simulink model "turbo_controller"  (R2025a)
settings: Solver=FixedStepAuto  StartTime=0.0  StopTime=inf  FixedStep=0.001  RelTol=1e-3
PostLoadFcn:
  | % 自动定位同目录CubeMX文件；不需要外部初始化脚本。
  | codertarget.data.setParameterValue('turbo_controller','STM32CubeMX.ProjectFile',fullfile(fileparts(get_param('turbo_controller','FileName')),'turbo_f407.ioc'));
InitFcn:
  | % 中文说明：按原控制器字段与类型创建三组接口总线；控制参数已内嵌。
  | tc_names=["EValve_Cycle" "EValve_Open" "Eblast_Cycle" "Eblast_Open" "Motor_Cycle" "Motor_Open" "EValve_Enable" "Eblast_Enable" "Motor_Enable" "SWO_Firework" "SWO_BleedAir" "EngineState" "Flag_ECUReset_Clear" "Flag_ECUReset_Save" "Flag_Reset_Enable" "Accelerator" "Nc_dem" "Nc"]; tc_types=["uint16" "uint16" "uint16" "uint16" "uint16" "uint16" "uint8" "uint8" "uint8" "uint8" "uint8" "uint8" "uint8" "uint8" "uint8" "single" "single" "single"];
  | for tc_k=1:numel(tc_names)
  |  tc_e(tc_k)=Simulink.BusElement; tc_e(tc_k).Name=char(tc_names(tc_k)); tc_e(tc_k).DataType=char(tc_types(tc_k));
  | end
  | EngineControl_Out=Simulink.Bus; EngineControl_Out.DataScope='Exported'; EngineControl_Out.Elements=tc_e;
  | clear tc_e tc_names tc_types tc_k
  | tc_names=["savedata1" "savedata2" "savedata3" "savedata4" "savedata5" "savedata6" "savedata7" "savedata8" "savedata9" "savedata10" "savedata11" "savedata12" "savedata13" "savedata14" "savedata15" "savedata16" "savedata17" "savedata18" "savedata19" "savedata20" "savedata21" "savedata22" "savedata23" "savedata24" "savedata25"]; tc_types=["single" "single" "single" "single" "single" "single" "single" "single" "single" "single" "single" "single" "single" "single" "single" "single" "single" "single" "single" "single" "single" "single" "single" "single" "single"];
  | for tc_k=1:numel(tc_names)
  |  tc_e(tc_k)=Simulink.BusElement; tc_e(tc_k).Name=char(tc_names(tc_k)); tc_e(tc_k).DataType=char(tc_types(tc_k));
  | end
  | SaveData_Out=Simulink.Bus; SaveData_Out.DataScope='Exported'; SaveData_Out.Elements=tc_e;
  | clear tc_e tc_names tc_types tc_k
  | tc_names=["senddata1" "senddata2" "senddata3" "senddata4" "senddata5" "senddata6" "senddata7" "senddata8" "senddata9" "senddata10" "senddata11" "senddata12" "senddata13" "senddata14" "senddata15" "senddata16" "senddata17" "senddata18" "senddata19" "senddata20" "senddata21" "senddata22" "senddata23" "senddata24" "senddata25" "senddata26" "senddata27" "senddata28" "senddata29"]; tc_types=["uint8" "uint8" "uint8" "uint8" "uint8" "uint8" "uint8" "uint8" "uint8" "uint8" "uint8" "uint8" "uint8" "uint8" "uint8" "uint8" "uint8" "uint8" "uint8" "uint8" "uint8" "uint8" "uint8" "uint8" "uint8" "uint8" "uint8" "uint8" "uint8"];
  | for tc_k=1:numel(tc_names)
  |  tc_e(tc_k)=Simulink.BusElement; tc_e(tc_k).Name=char(tc_names(tc_k)); tc_e(tc_k).DataType=char(tc_types(tc_k));
  | end
  | SendData_Out=Simulink.Bus; SendData_Out.DataScope='Exported'; SendData_Out.Elements=tc_e;
  | clear tc_e tc_names tc_types tc_k
  | 
  | % 以下为接口中文说明；只设置描述，不改变数值或数据类型。
  | EngineControl_Out.Description='执行控制输出（阀、电机、点火、状态及复位请求）';
  | tc_cn=["EValve_Cycle（主油阀周期计数（每计数2毫秒））" "EValve_Open（主油阀开通计数（每计数2毫秒））" "Eblast_Cycle（副油阀周期计数（每计数2毫秒））" "Eblast_Open（副油阀开通计数（每计数2毫秒））" "Motor_Cycle（起动电机周期计数）" "Motor_Open（起动电机开通计数）" "EValve_Enable（主油阀驱动使能）" "Eblast_Enable（副油阀驱动使能）" "Motor_Enable（起动电机使能）" "SWO_Firework（点火器使能（1开））" "SWO_BleedAir（引气阀使能（1开））" "EngineState（发动机状态）" "Flag_ECUReset_Clear（清除复位恢复状态请求）" "Flag_ECUReset_Save（保存复位恢复数据请求）" "Flag_Reset_Enable（处理器软件复位请求）" "Accelerator（油门／油泵给定控制量）" "Nc_dem（控制目标转速）" "Nc（发动机反馈转速（转每分））"];
  | tc_elements=EngineControl_Out.Elements;
  | for tc_k=1:numel(tc_cn)
  |  tc_elements(tc_k).Description=char(tc_cn(tc_k));
  | end
  | EngineControl_Out.Elements=tc_elements;
  | clear tc_cn tc_elements tc_k
  | SaveData_Out.Description='25项运行记录；字段含义按当前模型数据来源解释';
  | tc_cn=["savedata1（指令回显记录）" "savedata2（入口总温记录（℃））" "savedata3（电源电压记录）" "savedata4（排气温度记录（℃））" "savedata5（标定燃油压力记录）" "savedata6（副油阀占空比记录（％））" "savedata7（主油阀占空比记录（％））" "savedata8（温度修正转速记录）" "savedata9（开关输出及反馈位域）" "savedata10（物理转速记录）" "savedata11（油泵目标给定原始值）" "savedata12（起动电机占空比记录（％））" "savedata13（发动机状态码记录）" "savedata14（故障告警位域记录）" "savedata15（模型记录帧序号）" "savedata16（处理器温度记录（℃））" "savedata17（装订转速记录（沿用旧电源字段名））" "savedata18（导航高度记录）" "savedata19（飞行空速记录）" "savedata20（主阀旧记录位（恒零保留））" "savedata21（第21项保留记录（恒零））" "savedata22（保留记录项22）" "savedata23（保留记录项23）" "savedata24（保留记录项24）" "savedata25（保留记录项25）"];
  | tc_elements=SaveData_Out.Elements;
  | for tc_k=1:numel(tc_cn)
  |  tc_elements(tc_k).Description=char(tc_cn(tc_k));
  | end
  | SaveData_Out.Elements=tc_elements;
  | clear tc_cn tc_elements tc_k
  | SendData_Out.Description='29字段回传及外设命令接口；板端上位机帧只取第3至27字段';
  | tc_cn=["senddata1（回传发送允许标志（不直接上线路））" "senddata2（回传载荷长度25字节）" "senddata3（回传指令回显字节）" "senddata4（总温编码字节（℃＋80））" "senddata5（电源电压编码字节）" "senddata6（排温编码高字节）" "senddata7（排温编码低字节）" "senddata8（燃油压力编码高字节）" "senddata9（燃油压力编码低字节）" "senddata10（副油阀占空比字节（％））" "senddata11（主油阀占空比字节（％））" "senddata12（修正转速编码高字节）" "senddata13（修正转速编码低字节）" "senddata14（驱动及反馈状态位域）" "senddata15（物理转速编码高字节）" "senddata16（物理转速编码低字节）" "senddata17（油泵目标给定高字节（串口二使用））" "senddata18（油泵目标给定低字节（串口二使用））" "senddata19（起动电机占空比命令（串口一使用））" "senddata20（发动机状态码字节）" "senddata21（故障告警位域字节）" "senddata22（帧序号占位（板端另行填写））" "senddata23（处理器温度编码（℃＋50））" "senddata24（控制目标转速编码高字节）" "senddata25（控制目标转速编码低字节）" "senddata26（占位字节（板端改填实测泵速高字节））" "senddata27（占位字节（板端改填实测泵速低字节））" "senddata28（装订转速高字节（本板未发送））" "senddata29（装订转速低字节（本板未发送））"];
  | tc_elements=SendData_Out.Elements;
  | for tc_k=1:numel(tc_cn)
  |  tc_elements(tc_k).Description=char(tc_cn(tc_k));
  | end
  | SendData_Out.Elements=tc_elements;
  | clear tc_cn tc_elements tc_k
  | 
  | 
  | % FRAM模块化事务：接口类型和上电初始状态，随模型保存，无外部初始化文件。
  | clear FM_elements
  | FM_elements(1)=Simulink.BusElement;FM_elements(1).Name='phase';FM_elements(1).DataType='uint8';FM_elements(1).Dimensions=[1 1];FM_elements(1).Description='phase（当前事务阶段）';
  | FM_elements(2)=Simulink.BusElement;FM_elements(2).Name='a';FM_elements(2).DataType='uint8';FM_elements(2).Dimensions=[64 1];FM_elements(2).Description='a（启动时缓存的首区64字节）';
  | FM_elements(3)=Simulink.BusElement;FM_elements(3).Name='active';FM_elements(3).DataType='uint16';FM_elements(3).Dimensions=[1 1];FM_elements(3).Description='active（当前有效记录区地址）';
  | FM_elements(4)=Simulink.BusElement;FM_elements(4).Name='generation';FM_elements(4).DataType='uint32';FM_elements(4).Dimensions=[1 1];FM_elements(4).Description='generation（当前有效记录代号）';
  | FM_elements(5)=Simulink.BusElement;FM_elements(5).Name='record';FM_elements(5).DataType='uint8';FM_elements(5).Dimensions=[64 1];FM_elements(5).Description='record（本次冻结的待写记录）';
  | FM_elements(6)=Simulink.BusElement;FM_elements(6).Name='addr';FM_elements(6).DataType='uint16';FM_elements(6).Dimensions=[1 1];FM_elements(6).Description='addr（本次备用写入地址）';
  | FM_elements(7)=Simulink.BusElement;FM_elements(7).Name='lastSave';FM_elements(7).DataType='single';FM_elements(7).Dimensions=[1 1];FM_elements(7).Description='lastSave（上次开始保存的秒数）';
  | FM_elements(8)=Simulink.BusElement;FM_elements(8).Name='lastState';FM_elements(8).DataType='uint8';FM_elements(8).Dimensions=[1 1];FM_elements(8).Description='lastState（上次保存时的发动机状态）';
  | FM_elements(9)=Simulink.BusElement;FM_elements(9).Name='boot';FM_elements(9).DataType='boolean';FM_elements(9).Dimensions=[1 1];FM_elements(9).Description='boot（启动记录是否允许恢复）';
  | FM_elements(10)=Simulink.BusElement;FM_elements(10).Name='consumed';FM_elements(10).DataType='boolean';FM_elements(10).Dimensions=[1 1];FM_elements(10).Description='consumed（本次启动恢复通知是否已发送）';
  | FM_elements(11)=Simulink.BusElement;FM_elements(11).Name='payload';FM_elements(11).DataType='uint8';FM_elements(11).Dimensions=[20 1];FM_elements(11).Description='payload（当前20字节恢复内容）';
  | ... (+35 lines)
model workspace (MAT data in the model file):
  CRC16_Table_Reference = [0 4129 8258 12387 16516 20645 24774 28903 33032 37161 41290 45419 ... (256 elements, 256x1)]
  PE_Kaer = [0.15402 0.15402 0.12264 0.10076 0.09481 0.07601 0.07111 0.0569 0.05198 0.04926 0.05308 0.04325 ... (13 elements, 1x13)]
  PE_Nr = [21.2982 61.4260372 67.7475458 72.7394382 76.845934 80.6988798 83.8449282 86.6491912 88.9382406 89.178606 91.1938214 93.4068058 ... (13 elements, 1x13)]
  PE_Pump_Translate = 33.5999984741
  PE_RotaSpeed_Translate = 860
  PE_Taer = [0.4939154 0.4939154 0.40780982 0.34066978 0.31622756 0.30405716 0.34300244 0.26785022 0.37393554 0.23914836 0.44563948 0.31044662 ... (13 elements, 1x13)]
  PF_ACCFULLRANGE = 3360
  PF_Flag_ECUReset = 0
  PF_Flag_rx_suc = 1
  PF_Gear_Info = [40000; 45000; 50000; 55000; 57000; 59000; 60000; 61000; 61000; 61000; 61000; 61000]
  PF_K_TiaoJie = 1
  PF_Kpu = 10
  PF_MySet_Rxdata = [0 0 0 0 0 0 0 0 0 0 0 0 ... (50 elements, 50x1)]
  PF_MyUsart1_Rxdata = [0 0 0 0 0 0 0 0 0 0 0 0 ... (50 elements, 50x1)]
  PF_MyUsart2_Rxdata = [0 0 0 0 0 0 0 0 0 0 0 0 ... (50 elements, 50x1)]
  PF_Reset_Information = [0 0 0 0 0 0 0 0 0 0 0 0 ... (20 elements, 20x1)]
  PF_Sensor_X1_T4 = [0 4095]
  PF_Sensor_X2_T4 = [0 1.66666698456]
  PF_Sensor_X3_T4 = [0 504 999 1497 2010 2529 3051 3568 4076 4571 4959]
  PF_Sensor_X_P2 = [0.5 3]
  PF_Sensor_X_Poil = [0.5 3]
  PF_Sensor_X_T1t = [-50 300]
  PF_Sensor_X_Vpower = [0 3]
  PF_Sensor_X_Vpump = [0 3]
  PF_Sensor_Y1_T4 = [0 3]
  PF_Sensor_Y2_T4 = [0 5000]
  PF_Sensor_Y3_T4 = [0 100 200 300 400 500 600 700 800 900 980]
  PF_Sensor_Y_P2 = [0 1000]
  PF_Sensor_Y_Poil = [0 1000]
  PF_Sensor_Y_T1t = [-50 300]
  PF_Sensor_Y_Vpower = [0 33]
  PF_Sensor_Y_Vpump = [0 33]
  PG_CtrlMode_CloseLoop : mpt.Parameter (value not decoded)
  PG_CtrlMode_ManualAcc : mpt.Parameter (value not decoded)
  PG_CtrlMode_Origin : mpt.Parameter (value not decoded)
  PG_CtrlMode_Start : mpt.Parameter (value not decoded)
  PG_CtrlMode_Stop : mpt.Parameter (value not decoded)
  PG_ES_Clp : mpt.Parameter (value not decoded)
  PG_ES_EngStart : mpt.Parameter (value not decoded)
  PG_ES_Manual : mpt.Parameter (value not decoded)
  PG_ES_Origin : mpt.Parameter (value not decoded)
  PG_ES_Stop : mpt.Parameter (value not decoded)
  PG_Instr_BleedAirSet : mpt.Parameter (value not decoded)
  PG_Instr_CloseLoop : mpt.Parameter (value not decoded)
  PG_Instr_ECUReSet : mpt.Parameter (value not decoded)
  PG_Instr_EValveSet : mpt.Parameter (value not decoded)
  PG_Instr_EblastSet : mpt.Parameter (value not decoded)
  PG_Instr_Erase : mpt.Parameter (value not decoded)
  PG_Instr_FireWorkSet : mpt.Parameter (value not decoded)
  PG_Instr_ManualPlus : mpt.Parameter (value not decoded)
  PG_Instr_ManualrReduce : mpt.Parameter (value not decoded)
  PG_Instr_MotorSet : mpt.Parameter (value not decoded)
  PG_Instr_OilSet : mpt.Parameter (value not decoded)
  PG_Instr_SelfCheck : mpt.Parameter (value not decoded)
  PG_Instr_Start : mpt.Parameter (value not decoded)
  PG_Instr_Stop : mpt.Parameter (value not decoded)
  PG_Instr_StopZero : Simulink.Parameter (value not decoded)
  PG_Location_Air : Simulink.Parameter (value not decoded)
  PG_Location_Gnd : Simulink.Parameter (value not decoded)
  PG_ServoCtrlMode_CloseLoop : Simulink.Parameter (value not decoded)
  PG_ServoCtrlMode_CloseLoopMax : Simulink.Parameter (value not decoded)
  PG_ServoCtrlMode_CloseLoopMin : Simulink.Parameter (value not decoded)
  PG_ServoCtrlMode_ManualAcc : Simulink.Parameter (value not decoded)
  PG_ServoCtrlMode_ManualAccMax : Simulink.Parameter (value not decoded)
  PG_ServoCtrlMode_ManualAccMin : Simulink.Parameter (value not decoded)
  PG_SpeedDot_Permit : Simulink.Parameter (value not decoded)
  PL_EngineModel_Actuator = [0 10 100]
  PL_EngineModel_EngineStar_Press_P2 = [1013 1098.4 1099.144828 1099.931034 1103.613793 1162.662069 1143.793103 1131.006897 1123.186207 1117.6 1114 1111.806897 ... (127 elements, 1x127)]
  PL_EngineModel_EngineStar_RotaSpeed = [200 2000 9584 9660 10220 10240 10260 10288 10308 10368 10380 10408 ... (127 elements, 1x127)]
  PL_EngineModel_EngineStar_Temp_Exhaust = [128 129 129.1 130 131 131.1 132 133 134 134.1 135 135.1 ... (127 elements, 1x127)]
  PL_EngineModel_EngineStar_Time = [0.05 0.1 0.15 0.2 0.25 0.3 0.35 0.4 0.45 0.5 0.55 0.6 ... (127 elements, 1x127)]
  PL_EngineModel_IdleAbove_Nr = [0 21.2982 61.4260372 67.7475458 72.7394382 76.845934 80.6988798 83.8449282 86.6491912 88.9382406 89.178606 91.1938214 ... (14 elements, 1x14)]
  PL_EngineModel_IdleAbove_P2r = [0.986923266716 1.57907722675 1.81593881076 1.99358499877 2.23044658278 2.43770046879 2.65482358747 2.84233900814 3.03972366149 3.18776215149 3.25684678016 3.3950160375 ... (14 elements, 1x14)]
  PL_EngineModel_IdleAbove_Tempr = [0.0536001429337 1.07200285867 1.63301768805 1.63659103091 1.66875111667 1.72592460247 1.77595140254 1.86171163123 1.95461854565 2.03323208862 2.03323208862 2.13685903162 ... (14 elements, 1x14)]
  PL_EngineModel_IdleAbove_Ter = [0.42434128 0.42434128 0.42434128 0.30669408 0.23570008 0.22150128 0.1997974 0.23803274 0.16115638 0.24279948 0.13600422 0.31308354 ... (14 elements, 1x14)]
  PL_EngineModel_IdleAbove_Wfr = [0 10.142 23.8337 27.8905 31.9473 36.0041 40.0609 44.1177 48.1745 52.2313 52.7384 56.7952 ... (14 elements, 1x14)]
  PL_EngineModel_Press_P2 = [400 400 400 400 400 400 400 400 400 400]
  PL_EngineModel_Rotaspeed = [0 20000 96400]
  PL_EngineModel_Temp_Exhaust = [500 500 500 500 500 500 500 500 500 500]
  PL_Kaer = [0.1 0.1 0.1 0.1 0.1 0.1]
  PL_Nr = [50 60 70 80 90 100]
  PL_Taer = [0.1 0.1 0.1 0.1 0.1 0.1]
  Sig : Simulink.Signal (value not decoded)
  Ts_ms : Simulink.Parameter (value not decoded)
  false : Simulink.Parameter (value not decoded)
  true : Simulink.Parameter (value not decoded)
symbols that are objects in the model workspace (value not decoded): PG_CtrlMode_CloseLoop, PG_CtrlMode_ManualAcc, PG_CtrlMode_Origin, PG_CtrlMode_Start, PG_CtrlMode_Stop, PG_ES_Clp, PG_ES_EngStart, PG_ES_Manual, PG_ES_Origin, PG_ES_Stop, PG_Instr_BleedAirSet, PG_Instr_CloseLoop, PG_Instr_EblastSet, PG_Instr_ECUReSet, PG_Instr_Erase, PG_Instr_EValveSet, PG_Instr_FireWorkSet, PG_Instr_ManualPlus, PG_Instr_ManualrReduce, PG_Instr_MotorSet, PG_Instr_OilSet, PG_Instr_SelfCheck, PG_Instr_Start, PG_Instr_Stop, PG_Instr_StopZero, PG_ServoCtrlMode_CloseLoop, PG_ServoCtrlMode_CloseLoopMax, PG_ServoCtrlMode_CloseLoopMin, PG_ServoCtrlMode_ManualAcc, PG_ServoCtrlMode_ManualAccMax, PG_ServoCtrlMode_ManualAccMin, Ts_ms
libraries: simulink x97, stm32blockslib x10, stm32f4xxblockslib x8
(part 26 of 26)

== stateflow chart turbo_controller/CLM/ClpControl/Aim__Parameter_Calculate/Aim_AccMaxMin_Cal1/HoldFirst/M_Rate_Limiter ==
  note: 目标转速怎样逐次接近装订值
      |
      | 输入Nc_Initial是进入时锁存的反馈转速，S_Dem_SpeedLoad是上位机要求。第一次先令受限目标等于
      | 初值，再根据目标在初值上方还是下方，记住上升或下降阶段。
      |
      | 上升时每次图表调用加140；下降时每次减100。若本次跨过装订目标，就直接取装订目标并进入跟随阶
      | 段。后续需求再次改变，仍按同样上升/下降步长逼近。
      | 可写成上升：新目标=min(旧目标+140,需求)；下降：新目标=max(旧目标-100,需求)。
      |
      | 例如40000升到40500，输出约40140、40280、40420、40500，最后一步不是40560。每次调用的140/100
      | 是转速增量，不是每秒的变化率；按20 ms有效调用折算才有每秒意义。
      |
      | 结果送父级形成Nc_dem，不直接改变实际转速，也不直接生成油泵给定。
  (default) -> (junction 26)
    settings: description=无附加条件的迁移路径，执行次序1；沿本图当前连接推进。
  (junction 26) -> (junction 3) [order 1] : [Start_A/*起动阶段或中间量编号*/== true/*真值*/]
    settings: description=本路径的判据/动作：[Start_A== true]。执行次序1；条件成立才执行本箭头动作。
  (junction 3) -> (junction 86) [order 1] : [S_Dem_SpeedLoad/*目标需求速度或转速负载或装订值*/>=Nc_Initial/*控制器转速变量初始*/]
    settings: description=本路径的判据/动作：[S_Dem_SpeedLoad>=Nc_Initial]。执行次序1；条件成立才执行本箭头动作。
  (junction 26) -> (junction 43) [order 2]
    settings: description=无附加条件的迁移路径，执行次序2；沿本图当前连接推进。
  (junction 3) -> (junction 55) [order 2] : {Start_A/*起动阶段或中间量编号*/ = false/*假值*/;
      | S_Dem_SpeedLoad_Limiter/*目标需求速度或转速负载或装订值限制器*/=Nc_Initial/*控制器转速变量初始*/;
      | Start_C/*起动条件输入或阶段编号*/= true/*真值*/;}
    settings: description=本路径的判据/动作：{Start_A = false; S_Dem_SpeedLoad_Limiter=Nc_Initial; Start_C= true;}。执行次序2；条件成立才执行本箭头动作。
  (junction 86) -> (junction 88) : {Start_A/*起动阶段或中间量编号*/ = false/*假值*/;
      | S_Dem_SpeedLoad_Limiter/*目标需求速度或转速负载或装订值限制器*/=Nc_Initial/*控制器转速变量初始*/;
      | Start_B/*起动阶段或中间量编号*/= true/*真值*/;}
    settings: description=本路径的判据/动作：{Start_A = false; S_Dem_SpeedLoad_Limiter=Nc_Initial; Start_B= true;}。执行次序1；条件成立才执行本箭头动作。
  (junction 55) -> (junction 43)
    settings: description=无附加条件的迁移路径，执行次序1；沿本图当前连接推进。
  (junction 88) -> (junction 55)
    settings: description=无附加条件的迁移路径，执行次序1；沿本图当前连接推进。
  (junction 43) -> (junction 71)
    settings: description=无附加条件的迁移路径，执行次序1；沿本图当前连接推进。
  (junction 71) -> (junction 94) [order 1] : [Start_B/*起动阶段或中间量编号*/== true/*真值*/]
    settings: description=本路径的判据/动作：[Start_B== true]。执行次序1；条件成立才执行本箭头动作。
  (junction 71) -> (junction 106) [order 2]
    settings: description=无附加条件的迁移路径，执行次序2；沿本图当前连接推进。
  (junction 94) -> (junction 95) : {S_Dem_SpeedLoad_Limiter/*目标需求速度或转速负载或装订值限制器*/=S_Dem_SpeedLoad_Limiter/*目标需求速度或转速负载或装订值限制器*/+140.0;}
    settings: description=本路径的判据/动作：{S_Dem_SpeedLoad_Limiter=S_Dem_SpeedLoad_Limiter+140.0;}。执行次序1；条件成立才执行本箭头动作。
  (junction 95) -> (junction 99) [order 1] : [S_Dem_SpeedLoad_Limiter/*目标需求速度或转速负载或装订值限制器*/>=S_Dem_SpeedLoad/*目标需求速度或转速负载或装订值*/]
    settings: description=本路径的判据/动作：[S_Dem_SpeedLoad_Limiter>=S_Dem_SpeedLoad]。执行次序1；条件成立才执行本箭头动作。
  (junction 95) -> (junction 103) [order 2]
    settings: description=无附加条件的迁移路径，执行次序2；沿本图当前连接推进。
  (junction 99) -> (junction 96) : {Start_B/*起动阶段或中间量编号*/ = false/*假值*/;
      | S_Dem_SpeedLoad_Limiter/*目标需求速度或转速负载或装订值限制器*/=S_Dem_SpeedLoad/*目标需求速度或转速负载或装订值*/;
      | Start_D/*起动阶段或中间量编号*/= true/*真值*/;}
    settings: description=本路径的判据/动作：{Start_B = false; S_Dem_SpeedLoad_Limiter=S_Dem_SpeedLoad; Start_D= true;}。执行次序1；条件成立才执行本箭头动作。
  (junction 103) -> (junction 106)
    settings: description=无附加条件的迁移路径，执行次序1；沿本图当前连接推进。
  (junction 96) -> (junction 103)
    settings: description=无附加条件的迁移路径，执行次序1；沿本图当前连接推进。
  (junction 106) -> (junction 121)
    settings: description=无附加条件的迁移路径，执行次序1；沿本图当前连接推进。
  (junction 121) -> (junction 116) [order 1] : [Start_C/*起动条件输入或阶段编号*/== true/*真值*/]
    settings: description=本路径的判据/动作：[Start_C== true]。执行次序1；条件成立才执行本箭头动作。
  (junction 121) -> (junction 123) [order 2]
    settings: description=无附加条件的迁移路径，执行次序2；沿本图当前连接推进。
  (junction 116) -> (junction 119) : {S_Dem_SpeedLoad_Limiter/*目标需求速度或转速负载或装订值限制器*/=S_Dem_SpeedLoad_Limiter/*目标需求速度或转速负载或装订值限制器*/-100.0;}
    settings: description=本路径的判据/动作：{S_Dem_SpeedLoad_Limiter=S_Dem_SpeedLoad_Limiter-100.0;}。执行次序1；条件成立才执行本箭头动作。
  (junction 119) -> (junction 111) [order 1] : [S_Dem_SpeedLoad_Limiter/*目标需求速度或转速负载或装订值限制器*/<=S_Dem_SpeedLoad/*目标需求速度或转速负载或装订值*/]
    settings: description=本路径的判据/动作：[S_Dem_SpeedLoad_Limiter<=S_Dem_SpeedLoad]。执行次序1；条件成立才执行本箭头动作。
  (junction 119) -> (junction 115) [order 2]
    settings: description=无附加条件的迁移路径，执行次序2；沿本图当前连接推进。
  (junction 111) -> (junction 120) : {Start_C/*起动条件输入或阶段编号*/ = false/*假值*/;
      | S_Dem_SpeedLoad_Limiter/*目标需求速度或转速负载或装订值限制器*/=S_Dem_SpeedLoad/*目标需求速度或转速负载或装订值*/;
      | Start_D/*起动阶段或中间量编号*/= true/*真值*/;}
    settings: description=本路径的判据/动作：{Start_C = false; S_Dem_SpeedLoad_Limiter=S_Dem_SpeedLoad; Start_D= true;}。执行次序1；条件成立才执行本箭头动作。
  (junction 115) -> (junction 123)
    settings: description=无附加条件的迁移路径，执行次序1；沿本图当前连接推进。
  (junction 120) -> (junction 115)
    settings: description=无附加条件的迁移路径，执行次序1；沿本图当前连接推进。
  (junction 123) -> (junction 128)
    settings: description=无附加条件的迁移路径，执行次序1；沿本图当前连接推进。
  (junction 128) -> (junction 127) [order 1] : [Start_D/*起动阶段或中间量编号*/== true/*真值*/]
    settings: description=本路径的判据/动作：[Start_D== true]。执行次序1；条件成立才执行本箭头动作。
  (junction 127) -> (junction 132) [order 1] : [S_Dem_SpeedLoad/*目标需求速度或转速负载或装订值*/>=S_Dem_SpeedLoad_Limiter/*目标需求速度或转速负载或装订值限制器*/]
    settings: description=本路径的判据/动作：[S_Dem_SpeedLoad>=S_Dem_SpeedLoad_Limiter]。执行次序1；条件成立才执行本箭头动作。
  (junction 128) -> (junction 137) [order 2]
    settings: description=无附加条件的迁移路径，执行次序2；沿本图当前连接推进。
  (junction 127) -> (junction 136) [order 2] : {S_Dem_SpeedLoad_Limiter/*目标需求速度或转速负载或装订值限制器*/=S_Dem_SpeedLoad_Limiter/*目标需求速度或转速负载或装订值限制器*/-100.0;}
    settings: description=本路径的判据/动作：{S_Dem_SpeedLoad_Limiter=S_Dem_SpeedLoad_Limiter-100.0;}。执行次序2；条件成立才执行本箭头动作。
  (junction 132) -> (junction 134) : {S_Dem_SpeedLoad_Limiter/*目标需求速度或转速负载或装订值限制器*/=S_Dem_SpeedLoad_Limiter/*目标需求速度或转速负载或装订值限制器*/+140.0;}
    settings: description=本路径的判据/动作：{S_Dem_SpeedLoad_Limiter=S_Dem_SpeedLoad_Limiter+140.0;}。执行次序1；条件成立才执行本箭头动作。
  (junction 134) -> (junction 143) [order 1] : [S_Dem_SpeedLoad_Limiter/*目标需求速度或转速负载或装订值限制器*/>=S_Dem_SpeedLoad/*目标需求速度或转速负载或装订值*/]
    settings: description=本路径的判据/动作：[S_Dem_SpeedLoad_Limiter>=S_Dem_SpeedLoad]。执行次序1；条件成立才执行本箭头动作。
  (junction 136) -> (junction 150) [order 1] : [S_Dem_SpeedLoad_Limiter/*目标需求速度或转速负载或装订值限制器*/<=S_Dem_SpeedLoad/*目标需求速度或转速负载或装订值*/]
    settings: description=本路径的判据/动作：[S_Dem_SpeedLoad_Limiter<=S_Dem_SpeedLoad]。执行次序1；条件成立才执行本箭头动作。
  (junction 143) -> (junction 144) : {
      | S_Dem_SpeedLoad_Limiter/*目标需求速度或转速负载或装订值限制器*/=S_Dem_SpeedLoad/*目标需求速度或转速负载或装订值*/;
      | }
    settings: description=本路径的判据/动作：{ S_Dem_SpeedLoad_Limiter=S_Dem_SpeedLoad; }。执行次序1；条件成立才执行本箭头动作。
  (junction 150) -> (junction 151) : {
      | S_Dem_SpeedLoad_Limiter/*目标需求速度或转速负载或装订值限制器*/=S_Dem_SpeedLoad/*目标需求速度或转速负载或装订值*/;
      | }
    settings: description=本路径的判据/动作：{ S_Dem_SpeedLoad_Limiter=S_Dem_SpeedLoad; }。执行次序1；条件成立才执行本箭头动作。
  (junction 136) -> (junction 145) [order 2]
    settings: description=无附加条件的迁移路径，执行次序2；沿本图当前连接推进。
  (junction 134) -> (junction 138) [order 2]
    settings: description=无附加条件的迁移路径，执行次序2；沿本图当前连接推进。
  (junction 145) -> (junction 137)
    settings: description=无附加条件的迁移路径，执行次序1；沿本图当前连接推进。
  (junction 144) -> (junction 138)
    settings: description=无附加条件的迁移路径，执行次序1；沿本图当前连接推进。
  (junction 151) -> (junction 145)
    settings: description=无附加条件的迁移路径，执行次序1；沿本图当前连接推进。
  (junction 138) -> (junction 151)
    settings: description=无附加条件的迁移路径，执行次序1；沿本图当前连接推进。
  (junction 137) -> (junction 156)
    settings: description=无附加条件的迁移路径，执行次序1；沿本图当前连接推进。
  data: S_Dem_SpeedLoad_Limiter output single =0; Nc_Initial input single =0; S_Dem_SpeedLoad input single; Start_A local boolean =1; Start_B local boolean =0; Start_C local boolean =0; Start_D local boolean =0

== stateflow chart turbo_controller/FPM/Subsystem/Timmer_ms_Lock ==
  note: 持续异常达到时间门限后锁存故障
      |
      | 输入In为真或内部Flag_Lock已经为真时计数。计数严格大于Time_ms/Ts_ms后，置Out和Flag_Lock为真
      | 。锁存之后，即便外部In恢复为假，也继续维持故障状态，直到模型/图初始化。
      |
      | 父级Time_ms=10000、Ts_ms=20，门限500次调用，采用“>”判断。这样短暂测速异常先走临时保护，
      | 持续约10 s才进入长期故障策略。计数有上限，不无限累加。
  (default) -> (junction 26)
    settings: description=无附加条件的迁移路径，执行次序1；沿本图当前连接推进。
  (junction 26) -> (junction 3) [order 1] : [(true/*真值*/ == In/*输入*/) || (true/*真值*/ == Flag_Lock/*标志锁存*/)]
    settings: description=本路径的判据/动作：[(true == In) || (true == Flag_Lock)]。执行次序1；条件成立才执行本箭头动作。
  (junction 3) -> (junction 5) [order 1] : [Cnt/*计数器*/ >= uint32/*三十二位无符号整数*/(100000)]
    settings: description=本路径的判据/动作：[Cnt >= uint32(100000)]。执行次序1；条件成立才执行本箭头动作。
  (junction 26) -> (junction 43) [order 2] : {Cnt/*计数器*/ = 0;Out/*输出*/ = false/*假值*/;}
    settings: description=本路径的判据/动作：{Cnt = 0;Out = false;}。执行次序2；条件成立才执行本箭头动作。
  (junction 3) -> (junction 10) [order 2] : {Cnt/*计数器*/++;}
    settings: description=本路径的判据/动作：{Cnt++;}。执行次序2；条件成立才执行本箭头动作。
  (junction 5) -> (junction 12) : {Cnt/*计数器*/ = 100000;}
    settings: description=本路径的判据/动作：{Cnt = 100000;}。执行次序1；条件成立才执行本箭头动作。
  (junction 12) -> (junction 10)
    settings: description=无附加条件的迁移路径，执行次序1；沿本图当前连接推进。
  (junction 10) -> (junction 30)
    settings: description=无附加条件的迁移路径，执行次序1；沿本图当前连接推进。
  (junction 30) -> (junction 33) [order 1] : [Cnt/*计数器*/ >uint32/*三十二位无符号整数*/(Time_ms/*时间毫秒*//Ts_ms/*采样周期毫秒*/)]
    settings: description=本路径的判据/动作：[Cnt >uint32(Time_ms/Ts_ms)]。执行次序1；条件成立才执行本箭头动作。
  (junction 30) -> (junction 37) [order 2] : {Out/*输出*/ = false/*假值*/;}
    settings: description=本路径的判据/动作：{Out = false;}。执行次序2；条件成立才执行本箭头动作。
  (junction 33) -> (junction 36) : {Out/*输出*/ = true/*真值*/;
      | Flag_Lock/*标志锁存*/ = true/*真值*/;}
    settings: description=本路径的判据/动作：{Out = true; Flag_Lock = true;}。执行次序1；条件成立才执行本箭头动作。
  (junction 36) -> (junction 37)
    settings: description=无附加条件的迁移路径，执行次序1；沿本图当前连接推进。
  (junction 37) -> (junction 55)
    settings: description=无附加条件的迁移路径，执行次序1；沿本图当前连接推进。
  (junction 55) -> (junction 43)
    settings: description=无附加条件的迁移路径，执行次序1；沿本图当前连接推进。
  (junction 43) -> (junction 71)
    settings: description=无附加条件的迁移路径，执行次序1；沿本图当前连接推进。
  data: Cnt local uint32 =0; Out output boolean =0; In input boolean; Time_ms input single; Ts_ms parameter single; Flag_Lock local boolean =0

== matlab function turbo_controller/FRAM_复位恢复事务/Step01_Check（检查双区记录） ==
  data: state input; checked output Bus: FM_Checked size=1; rx input
function checked = CheckRecords(state, rx)
% 检查FRAM返回记录是否完整可信
% 
% SPI返回67字节，前3字节是命令/地址占位，后64字节才是记录。本步骤把首区缓存和本次返回的另一区分别检查，输出各区有效性、代号及20字节恢复内容。
% 
% 一条记录必须同时满足：前4字节为ECR1（69、67、82、49）；第64字节为165；第57～60字节的小端CRC32等于对第1～56字节重新计算的CRC32。只满足其中一项不算有效。
% 
% CRC32初值FFFFFFFF，每个输入字节与低位异或，再逐位右移，最低位为1时异或EDB88320，最后逐位取反。代号按小端还原：第1字节+第2字节×256+第3字节×65536+第4字节×16777216。
% 
% 本步骤只给检查结果，不决定哪条更新，也不修改FRAM。选择交给Step02，写后是否接受新记录交给Step05。
%#codegen
% 01：检查读回来的记录，只判断“数据靠不靠谱”，不决定控制动作。
% state（上一周期事务状态）：a 是启动时缓存的首区记录，phase 是当前阶段。
% rx（上一周期读回的67字节）：前3字节是命令头，后64字节才是记录。
% checked（检查结果）：有效标志、代号、恢复数据，以及本次原始记录。
% 只在启动选择或写后回读阶段计算CRC，避免每毫秒重复校验。
recordB = reshape(rx(4:67),64,1); % recordB（本次接收到的64字节）
checked = struct('validA',false,'validB',false, ...
 'generationA',uint32(0),'generationB',uint32(0), ...
 'payloadA',zeros(20,1,'uint8'),'payloadB',zeros(20,1,'uint8'), ...
 'recordB',recordB);
if state.phase == uint8(2) % 阶段2：两区均已读完，需要选择启动记录。
 checked.validA = RecordIsValid(state.a);
 checked.generationA = ReadLittle32(state.a(5:8));
 checked.payloadA = state.a(9:28);
end
if state.phase == uint8(2) || state.phase == uint8(17)
 % 阶段17：刚完成一次写入，只校验本次回读的备用区。
 checked.validB = RecordIsValid(recordB);
 checked.generationB = ReadLittle32(recordB(5:8));
 checked.payloadB = recordB(9:28);
end
end

function valid = RecordIsValid(record)
% valid（是否有效）：记录头、提交标志、CRC32三项必须同时正确。
% [69 67 82 49] 对应记录格式标识 ECR1（复位恢复记录第1版）。
valid = all(record(1:4)==uint8([69;67;82;49])) ...
 && record(64)==uint8(165) ...
 && ReadLittle32(record(57:60))==CalculateCRC32(record(1:56));
end

function value = ReadLittle32(bytes)
% value（32位整数）；bytes（低字节在前的4个字节）。
value=uint32(0);
for index=1:4 % index（字节序号）
 value=bitor(value,bitshift(uint32(bytes(index)),8*(index-1)));
end
end

function crc = CalculateCRC32(bytes)
% crc（CRC32校验值）：用于检测记录内容是否损坏。
% 反射多项式0xEDB88320；初值全1；处理结束后按位取反。
crc=uint32(4294967295);
for byteIndex=1:numel(bytes) % byteIndex（当前字节序号）
 crc=bitxor(crc,uint32(bytes(byteIndex)));
 for bitIndex=1:8 % bitIndex（当前字节内的比特序号）
  lowestBit=bitand(crc,uint32(1)); % lowestBit（最低位）
  crc=bitshift(crc,-1);
  if lowestBit~=0,crc=bitxor(crc,uint32(3988292384));end
 end
end
crc=bitcmp(crc);
end

== matlab function turbo_controller/FRAM_复位恢复事务/Step02_Select（选择启动恢复记录） ==
  data: checked input; startup output Bus: FM_Startup size=1
function startup = ChooseStartup(checked)
% 从双区中选出可用于启动恢复的一条
% 
% 两区都有效时比较记录代号，优先采用代号较大的一条；代号相同优先首区。只有一条有效就选该条；两条都无效则保持valid=false，不把随机字节用于恢复。
% 
% 输出包括所选区地址、代号和20字节内容。首区为512（0x0200），次区为768（0x0300）。代号表示保存先后，不是发动机转速或运行模式。
% 
% boot还要求所存状态字节为3或4才成立，这是记录恢复资格规则，不等于“所有有效记录都立即恢复”。后续Step05还要等待启动读取结束、20 ms边界且尚未通知，才发一次恢复通知。代号采用普通数值比较，没有在这里额外实现代号回绕后的新旧排序。
%#codegen
% 02：从两份已经检查过的记录中，挑出可以用于启动恢复的一份。
% checked（双区检查结果）由01模块提供；本模块不直接访问FRAM。
% startup（启动选择结果）：valid有效、active地址、generation代号、
% payload恢复内容、boot是否允许发出恢复通知。
startup=struct('valid',false,'active',uint16(768), ...
 'generation',uint32(0),'payload',zeros(20,1,'uint8'),'boot',false);
% 首区有效且不比次区旧时，选首区；代号相同时也优先选首区。
chooseA=checked.validA && (~checked.validB ...
 || checked.generationA>=checked.generationB); % chooseA（是否选首区）
if chooseA
 startup.valid=true;
 startup.active=uint16(512); % 首区地址0x0200。
 startup.generation=checked.generationA;
 startup.payload=checked.payloadA;
elseif checked.validB
 startup.valid=true;
 startup.active=uint16(768); % 次区地址0x0300。
 startup.generation=checked.generationB;
 startup.payload=checked.payloadB;
end
% 保存状态为3或4，才允许通知后面的控制逻辑进行复位恢复。
savedState=startup.payload(9); % savedState（保存的发动机状态）
startup.boot=startup.valid && (savedState==3 || savedState==4);
end

== matlab function turbo_controller/FRAM_复位恢复事务/Step03_Request（判断是否开始保存） ==
  data: state input; saveEvent output; control input; seconds input
function saveEvent = CheckSaveRequest(state, control, seconds)
% 判断这一拍是否可以开始新的保存事务
% 
% 先检查是否存在保存或清除请求：Flag_ECUReset_Save和Flag_ECUReset_Clear任一个非零都算有请求。再检查事务是否空闲，只有phase=10才允许开始，避免前一条尚未写完就覆盖快照。
% 
% 还要满足两个条件之一：距离上次开始保存至少0.5 s，或发动机模式与上次不同。计算为“当前秒数-上次保存秒数≥0.5”，时间单位是s，不是调用次数。
% 
% 例：刚保存0.1 s且模式未变，本拍不保存；已过0.5 s且有请求，可以保存；模式刚变且有请求，即使不足0.5 s也可以保存。输出saveEvent是一拍的开始许可，不代表FRAM已写成功。
%#codegen
% 03：只回答一个问题——“这一毫秒要不要开始保存？”
% state（事务状态）；control（执行控制总线）；seconds（当前秒数）。
% saveEvent（本周期开始保存）：只在空闲阶段10产生。
% 请求来自 Flag_ECUReset_Save（保存请求）或 Flag_ECUReset_Clear（清除请求）。
% 普通重复保存至少间隔0.5秒；发动机状态改变时允许提前保存。
hasRequest=control.Flag_ECUReset_Save~=0 ...
 || control.Flag_ECUReset_Clear~=0; % hasRequest（存在保存或清除请求）
intervalPassed=single(seconds)-state.lastSave>=single(0.5); % 保存间隔已到。
stateChanged=control.EngineState~=state.lastState; % 发动机状态发生改变。
saveEvent=state.phase==uint8(10) && hasRequest ...
 && (intervalPassed || stateChanged);
end

== matlab function turbo_controller/CLM/ClpControl/Fault_Process/D9-Nr-T5r ==
  data: u1 input; u2 input; xin1 input; yin1 input; xin2 input; yin2 input; xin3 input; yin3 input; y output
function y = interp2D(u1,u2,xin1,yin1,xin2,yin2,xin3,yin3) %利用转速（u1/rpm）、高度（u2/km）插值；function（函数）；y（输出）；interp2D（二维插值）；u1（输入一）；u2（输入二）；xin1（第一横坐标）；yin1（第一纵坐标）；xin2（第二横坐标）；yin2（第二纵坐标）；xin3（第三横坐标）；yin3（第三纵坐标）
% 按转速和高度插出备用油泵给定
% 
% 父级传入装订转速N、以km表示的高度H，以及三条高度层曲线的转速断点和给定表。每条曲线先用interp1按N线性插值，获得该高度层的给定；代码采用linear和extrap，超出转速断点时允许线性外推。
% 
% 随后再按高度插值：H<5 km时，在0与5 km曲线结果之间插；H>=5 km时，在5与10 km曲线结果之间插。
% 例如H=2.5 km，输出是0和5 km两条曲线给定的中点；H=7.5 km则取5和10 km结果的中点。
% 
% 公式可写为：
% 低层：u=u0+(u5-u0)×H/5；
% 高层：u=u5+(u10-u5)×(H-5)/5。
% 高度超出0～10 km时，公式仍会外推，并不自动按端点截住。
% 
% 输出是转速故障备用给定，先交父级GeneralFilter限制幅值和每次变化量，再由故障标志决定是否采用。它不是新增的温度测量，也不替代真实转速采集。
%#codegen

if u2<5 % if（如果）；u2（输入二）
    Point1 = interp1(xin1,yin1,u1,'linear','extrap'); % Point1（第一插值结果）；interp1（一维插值）；xin1（第一横坐标）；yin1（第一纵坐标）；u1（输入一）；linear（线性）；extrap（外推）
    Point2 = interp1(xin2,yin2,u1,'linear','extrap'); % Point2（第二插值结果）；interp1（一维插值）；xin2（第二横坐标）；yin2（第二纵坐标）；u1（输入一）；linear（线性）；extrap（外推）
    y = Point1 + (Point1 - Point2)/5*(0 - u2); % y（输出）；Point1（第一插值结果）；Point2（第二插值结果）；u2（输入二）
    
else % else（否则）
    Point1 = interp1(xin2,yin2,u1,'linear','extrap'); % Point1（第一插值结果）；interp1（一维插值）；xin2（第二横坐标）；yin2（第二纵坐标）；u1（输入一）；linear（线性）；extrap（外推）
    Point2 = interp1(xin3,yin3,u1,'linear','extrap'); % Point2（第二插值结果）；interp1（一维插值）；xin3（第三横坐标）；yin3（第三纵坐标）；u1（输入一）；linear（线性）；extrap（外推）
    y = Point1 + (Point1 - Point2)/5*(5 - u2); % y（输出）；Point1（第一插值结果）；Point2（第二插值结果）；u2（输入二）
end % end（结束）

if u2 <0 % if（如果）；u2（输入二）
    y=interp1(xin1,yin1,u1,'linear','extrap'); % y（输出）；interp1（一维插值）；xin1（第一横坐标）；yin1（第一纵坐标）；u1（输入一）；linear（线性）；extrap（外推）
end % end（结束）
if u2 >11 % if（如果）；u2（输入二）
    y=interp1(xin3,yin3,u1,'linear','extrap'); % y（输出）；interp1（一维插值）；xin3（第三横坐标）；yin3（第三纵坐标）；u1（输入一）；linear（线性）；extrap（外推）
end % end（结束）

== stateflow chart turbo_controller/CLM/ClpControl/Fault_Process/GeneralFilter/Range ==
  note: 本实例先把故障备份曲线给出的泵编码限制在父级的X_llim～X_ulim内，再送后续死区和每拍步长处理
      | 。它只做幅值限制；差值小于20保持、否则每拍加减10在父级完成。
      |
      | 把一个数限制在允许范围内
      |
      | 输入包括待处理值、允许下限和允许上限。先比较是否越过上限，越过就输出上限；未超过上限时再检
      | 查下限，小于下限就输出下限；落在范围内则原样通过。恰好等于边界的值也保留。
      |
      | 计算式：输出 = min(max(输入，下限)，上限)。
      | 例如下限为0、上限为100时，输入120输出100，输入-5输出0，输入60输出60。这里不做平均、不计算
      | 变化速度，也不记住上一拍；它只防止当前数值越界。具体边界由父子系统连入，不能把此处的输出一
      | 律理解为百分比。
  (default) -> (junction 6)
    settings: description=无附加条件的迁移路径，执行次序1；沿本图当前连接推进。
  (junction 6) -> (junction 7) [order 1] : [In/*输入*/ <= Min/*下限*/]
    settings: description=本路径的判据/动作：[In <= Min]。执行次序1；条件成立才执行本箭头动作。
  (junction 6) -> (junction 29) [order 2] : {Out/*输出*/ = In/*输入*/;}
    settings: description=本路径的判据/动作：{Out = In;}。执行次序2；条件成立才执行本箭头动作。
  (junction 7) -> (junction 11) : {Out/*输出*/ = Min/*下限*/;}
    settings: description=本路径的判据/动作：{Out = Min;}。执行次序1；条件成立才执行本箭头动作。
  (junction 11) -> (junction 29)
    settings: description=无附加条件的迁移路径，执行次序1；沿本图当前连接推进。
  (junction 29) -> (junction 13)
    settings: description=无附加条件的迁移路径，执行次序1；沿本图当前连接推进。
  (junction 13) -> (junction 15) [order 1] : [Out/*输出*/ >= Max/*上限*/]
    settings: description=本路径的判据/动作：[Out >= Max]。执行次序1；条件成立才执行本箭头动作。
  (junction 13) -> (junction 20) [order 2]
    settings: description=无附加条件的迁移路径，执行次序2；沿本图当前连接推进。
  (junction 15) -> (junction 17) : {Out/*输出*/ = Max/*上限*/;}
    settings: description=本路径的判据/动作：{Out = Max;}。执行次序1；条件成立才执行本箭头动作。
  (junction 17) -> (junction 20)
    settings: description=无附加条件的迁移路径，执行次序1；沿本图当前连接推进。
  (junction 20) -> (junction 25)
    settings: description=无附加条件的迁移路径，执行次序1；沿本图当前连接推进。
  data: In input single; Max input single; Min input single; Out output single =0

== matlab function turbo_controller/FRAM_复位恢复事务/Step04_Pack（打包本次运行记录） ==
  data: state input; payload output; control input; send input; data input; saveEvent input; record output
function [payload, record] = BuildRecord(state, control, send, data, saveEvent)
% 在开始保存时冻结关键运行量，打成带校验的记录
% 
% 只有saveEvent为真才打包；否则输出清零占位，后续由事务状态保持真正待写记录。先形成20字节恢复内容：1～2为AA55；7～8为泵给定高、低字节；9为发动机模式；10为命令回显；11～13为目标转速；14～16为实际转速；18为前17字节模256累加和，19为异或校验。其余未赋值字段保持0。
% 
% 泵给定先限制0～65535再拆两字节。转速用三字节高位在前，例如50000保存为0、195、80。目标来自data.savedata17，虽然记录层部分旧名称叫电源，这条线实际传的是通信目标SpeedLoad。清除请求将保存模式写0，使其失去恢复资格，并非物理擦空整片FRAM。
% 
% 再打成64字节外层记录：1～4为ECR1，5～8为新代号（旧代号+1，小端），9～28放20字节恢复内容，57～60为前56字节CRC32。最后提交字节先不置165，由Step06在完整写入后单独提交。
% 
% 这里仅生成字节数组，不执行SPI；同一次事务后续始终写这份冻结快照，避免不同阶段混入不同时刻的数据。
%#codegen
% 04：把运行状态整理成“20字节恢复内容”和“64字节完整记录”。
% state（上一周期状态）；control（执行控制）；send（回传协议）；
% data（运行记录总线）；saveEvent（本周期开始保存）。
% 本模块只组装数据，不操作SPI，也不推进事务阶段。
payload=zeros(20,1,'uint8'); % payload（20字节恢复内容）
record=zeros(64,1,'uint8'); % record（64字节完整记录）
if ~saveEvent,return;end % 没有开始保存时，不重复计算校验。

% 一、填写恢复内容。所有字段均明确转换成字节。
payload(1:2)=uint8([170;85]); % 恢复内容头：0xAA、0x55。
throttle=uint16(min(max(control.Accelerator,0),65535)); % throttle（限幅油门）
payload(7)=uint8(bitshift(throttle,-8)); % 油门高字节。
payload(8)=uint8(bitand(throttle,255)); % 油门低字节。
payload(9)=uint8(control.EngineState); % 发动机状态。
if control.Flag_ECUReset_Clear~=0
 payload(9)=uint8(0); % 清除恢复资格：保存状态置零，其余格式不变。
end
payload(10)=uint8(send.senddata3); % 回传指令回显字节。
demand=uint32(max(data.savedata17,0)); % demand（装订转速）
actual=uint32(max(control.Nc,0)); % actual（实际转速）
payload(11:13)=ToBig24(demand); % 3字节，高字节在前。
payload(14:16)=ToBig24(actual);
% 第3～6、17、20字节保留为零，保持原有恢复格式。

% 二、填写恢复内容自身的校验。
sumByte=uint8(0);xorByte=uint8(0); % sumByte（累加校验）；xorByte（异或校验）。
for index=1:17
 sumByte=uint8(mod(double(sumByte)+double(payload(index)),256));
 xorByte=bitxor(xorByte,payload(index));
end
payload(18)=sumByte;payload(19)=xorByte;

% 三、填写完整记录头、递增代号、恢复内容及CRC32。
record(1:4)=uint8([69;67;82;49]); % ECR1（复位恢复记录第1版）。
record(5:8)=ToLittle32(state.generation+uint32(1)); % 新代号，低字节在前。
record(9:28)=payload;
record(57:60)=ToLittle32(CalculateCRC32(record(1:56)));
% 第64字节暂时为0；必须等数据写完，再由06模块单独写165完成提交。
end

function bytes = ToBig24(value)
% bytes（3字节数组）；value（待编码整数）；保留最低24位。
bytes=uint8([bitand(bitshift(value,-16),255); ...
 bitand(bitshift(value,-8),255);bitand(value,255)]);
end

function bytes = ToLittle32(value)
% bytes（4字节数组）：低字节在前，用于记录代号和CRC值。
bytes=zeros(4,1,'uint8');
for index=1:4
 bytes(index)=uint8(bitand(bitshift(value,-8*(index-1)),255));
end
end

function crc = CalculateCRC32(bytes)
% CRC32（循环冗余校验）：算法与01模块保持一致，用于写后完整性核对。
crc=uint32(4294967295);
for byteIndex=1:numel(bytes)
 crc=bitxor(crc,uint32(bytes(byteIndex)));
 for bitIndex=1:8
  lowestBit=bitand(crc,uint32(1));
  crc=bitshift(crc,-1);
  if lowestBit~=0,crc=bitxor(crc,uint32(3988292384));end
 end
end
crc=bitcmp(crc);
end

== matlab function turbo_controller/FRAM_复位恢复事务/Step05_Update（推进事务并更新状态） ==
  data: state input; next output Bus: FM_State size=1; control input; seconds input; checked input; startup input; saveEvent input; payload input; record input; restore output; info output; errors output
function [next, restore, info, errors] = UpdateTransaction(state, control, seconds, checked, startup, saveEvent, payload, record)
% 每拍推进一个FRAM事务阶段，并保留必要记忆
% 
% 输入state是上一拍状态，next先完整复制它，本拍只修改当前阶段需要的字段。输出next经StateMemory延迟，下一拍才成为新的state；因此本步骤不是一次调用就完成全部SPI操作。
% 
% 启动阶段0→1→2：发首区读取后缓存返回，再读次区，采用Step02选出的有效记录，最后进入空闲10。
% 空闲10：saveEvent成立时，记住本次时间、模式、内容和完整记录；当前有效首区则选次区写，反之选首区，进入11。
% 写入11～17：先使备用区失效，再发写使能、完整记录、写使能、提交165、回读，最后等待并检查返回。具体命令由Step06按旧state生成，两者要配合阅读。
% 验证17：只有回读记录有效且代号等于原代号+1，才把新地址设为有效区并更新代号；否则失败计数加1，保留旧有效区。两种情况最终都回空闲10。
% 
% 恢复通知另行判断：启动读取完成、boot有效、尚未通知，且四舍五入后的毫秒时间整除20时，restore置1并锁住consumed，保证一次启动只通知一次。info输出保持的20字节内容，errors输出累计验证失败次数。阶段推进本身不等于硬件回读成功。
%#codegen
% 05：事务调度员。只更新状态，不组包、不计算CRC、不直接操作SPI。
% state（上一周期状态）由00状态记忆提供；next（下一周期状态）写回00。
% checked（01检查结果）；startup（02启动选择）；saveEvent（03保存事件）；
% payload、record（04准备的新数据）；control（控制总线）；seconds（当前秒数）。
% restore（仅一次的恢复通知）、info（20字节恢复信息）、errors（失败计数）。
% 阶段表：0读首区→1读次区→2选择→10等待请求；
% 11失效→12写使能→13写数据→14写使能→15提交→16回读→17核对。
next=state; % 默认保持旧状态，只有当前阶段需要的字段才修改。
restore=uint8(0); % 默认不发恢复脉冲。

switch state.phase
 case 0 % 06模块本周期发首区读取命令。
  next.phase=uint8(1);
 case 1 % 上周期首区数据已返回，先缓存，再等待次区读取结果。
  next.a=checked.recordB;
  next.phase=uint8(2);
 case 2 % 两区已读完，采用02模块的选择结果。
  if startup.valid
   next.active=startup.active;
   next.generation=startup.generation;
   next.payload=startup.payload;
   next.boot=startup.boot;
  end
  next.phase=uint8(10);
 case 10 % 空闲：03模块同意开始保存时，冻结本次待写数据。
  if saveEvent
   next.lastSave=single(seconds);
   next.lastState=uint8(control.EngineState);
   next.payload=payload;
   next.record=record;
   if state.active==uint16(512)
    next.addr=uint16(768); % 当前首区有效，本次写次区。
   else
    next.addr=uint16(512); % 当前次区有效，本次写首区。
   end
   next.phase=uint8(11);
  end
 case 11 % 已发出使备用区失效的单字节写入。
  next.phase=uint8(12);
 case 12 % 已发出数据写入前的写使能。
  next.phase=uint8(13);
 case 13 % 已发出64字节记录写入。
  next.phase=uint8(14);
 case 14 % 已发出提交前的写使能。
  next.phase=uint8(15);
 case 15 % 已发出提交标记165的写入。
  next.phase=uint8(16);
 case 16 % 已发出回读命令，等待下一周期返回。
  next.phase=uint8(17);
 case 17 % 记录有效且代号正确，才切换当前有效区。
  expectedGeneration=state.generation+uint32(1); % expectedGeneration（期望代号）
  if checked.validB && checked.generationB==expectedGeneration
   next.active=state.addr;
   next.generation=expectedGeneration;
  else
   next.failures=state.failures+uint32(1); % 保留原有效区，失败次数加一。
  end
  next.phase=uint8(10);
end

% 启动恢复通知只发一次，并对齐到20毫秒边界。
aligned20ms=mod(round(seconds*1000),20)==0; % aligned20ms（已到20毫秒边界）
if next.phase>=uint8(10) && next.boot && ~next.consumed && aligned20ms
 restore=uint8(1);
 next.consumed=true; % consumed（本次启动的恢复通知已经发过）
end
info=next.payload;
errors=next.failures;
end

== matlab function turbo_controller/FRAM_复位恢复事务/Step06_Command（生成分步读写命令） ==
  data: state input; tx67 output; saveEvent input; en67 output; tx4 output; en4 output; tx1 output; en1 output
function [tx67,en67,tx4,en4,tx1,en1] = BuildCommand(state, saveEvent)
% 把事务阶段翻译成实际SPI字节帧
% 
% 本步骤只看上一拍state和开始保存事件，不在内部推进阶段。三类输出分别是67字节完整帧、4字节单字节写帧、1字节写使能命令，并各带一个发送允许。长度不同对应三路执行接口，不能混用。
% 
% 启动phase0读0x0200，phase1读0x0300；phase11向备用区地址+63写0，使它暂时无效；phase13写64字节完整记录；phase15向地址+63写165，表示提交完成；phase16回读备用区。其他阶段对应发送允许为假。
% 
% 完整帧=[操作码,地址高字节,地址低字节,64字节]。读操作码03，后64字节发0以产生SPI时钟；写操作码02，后64字节为冻结记录。4字节帧=[02,地址高,地址低,数值]。1字节命令06用于写使能，在saveEvent、phase12、phase14发出。
% 
% 例如备用区0x0300，提交字节地址0x033F，提交帧为02 03 3F A5。写使能必须在相应写入前发出，不能把多个阶段当成一帧连在一起。SPI实际传输由外面的带使能子系统完成。
%#codegen
% 06：把当前事务阶段翻译成SPI命令；外面的官方SPI模块负责真正收发。
% state（上一周期状态）；saveEvent（本周期开始保存）。
% tx67/en67（67字节长帧/允许发送）；tx4/en4（4字节提交帧/允许发送）；
% tx1/en1（单字节写使能命令/允许发送）。没有使能时不会启动硬件传输。
tx67=zeros(67,1,'uint8');
tx4=zeros(4,1,'uint8');
tx1=uint8(6); % 0x06：FRAM写使能命令。
en67=false;en4=false;
en1=saveEvent || state.phase==uint8(12) || state.phase==uint8(14);

switch state.phase
 case 0 % 启动：读取首区0x0200。
  tx67=LongFrame(uint8(3),uint16(512),state.record);en67=true;
 case 1 % 启动：读取次区0x0300。
  tx67=LongFrame(uint8(3),uint16(768),state.record);en67=true;
 case 11 % 先把备用区最后一个字节写0，标记“尚未完成”。
  tx4=CommitFrame(state.addr+uint16(63),uint8(0));en4=true;
 case 13 % 写入已经冻结的64字节记录。
  tx67=LongFrame(uint8(2),state.addr,state.record);en67=true;
 case 15 % 最后单独写165，标记“记录已完整提交”。
  tx4=CommitFrame(state.addr+uint16(63),uint8(165));en4=true;
 case 16 % 重新读出刚写的区，交给01、05模块验证。
  tx67=LongFrame(uint8(3),state.addr,state.record);en67=true;
end
end

function frame = LongFrame(opcode,address,record)
% frame（67字节帧）=命令1字节＋地址2字节＋数据64字节。
% opcode（操作码）：3读、2写；address（FRAM地址）；record（待写记录）。
frame=zeros(67,1,'uint8');
frame(1)=opcode;
frame(2)=uint8(bitshift(address,-8));
frame(3)=uint8(bitand(address,255));
if opcode==uint8(2),frame(4:67)=record;end % 读操作只需发送零填充。
end

function frame = CommitFrame(address,value)
% frame（4字节帧）=写命令＋地址高字节＋地址低字节＋标记值。
frame=uint8([2;uint8(bitshift(address,-8));uint8(bitand(address,255));value]);
end
